simulink model "LunarLandingModel"  (R2023b)
settings: Solver=VariableStepAuto  StartTime=0.0  StopTime=10  RelTol=1e-3
values from neighbouring files (symbols this model uses):
  rf = paramat.rf    [Differential_Eq.m]    (also in control_law.m; extractparameters.m = 1740000; rk4_method.m)
libraries: simulink x1
settings Model: Creator=HUAWEI  LastModifiedBy=HUAWEI

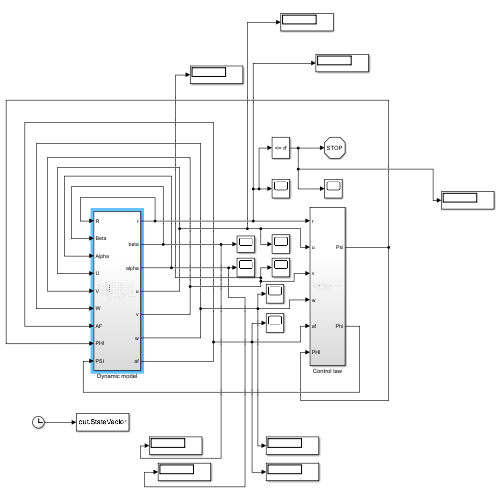
[thumbnail: Simulink's stored preview of the top-level diagram]
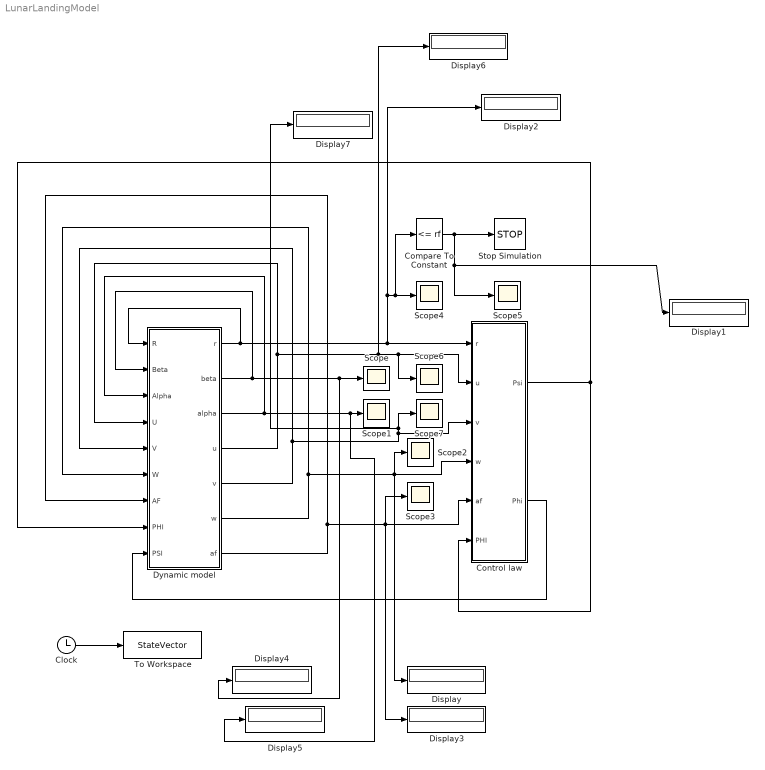
== system LunarLandingModel ==
  Clock : Clock
  Compare To Constant : simulink/Logic and Bit Operations/Compare To Constant  relop=<=  const=rf  OutDataTypeStr=boolean
  Control law : Subsystem
  Display{,1..7} (8 alike) : Display
  Dynamic model : Subsystem
  Scope{,1..7} (8 alike) : Scope
  Stop Simulation : Stop
  To Workspace : ToWorkspace  VariableName=StateVector  SaveFormat=Structure With Time  SampleTime=-1
  wires:
  Dynamic model/1(r) -> Dynamic model/1(R), Display2/1, Compare To Constant/1, Scope4/1, Control law/1(r)
  Dynamic model/2(beta) -> Dynamic model/2(Beta), Scope/1, Display4/1
  Dynamic model/3(alpha) -> Display5/1, Scope1/1, Dynamic model/3(Alpha)
  Compare To Constant/1 -> Scope5/1, Display1/1, Stop Simulation/1
  Clock/1 -> To Workspace/1
  Dynamic model/4(u) -> Control law/2(u), Scope6/1, Display6/1, Dynamic model/4(U)
  Dynamic model/5(v) -> Dynamic model/5(V), Display7/1, Scope7/1, Control law/3(v)
  Dynamic model/6(w) -> Dynamic model/6(W), Display/1, Scope2/1, Control law/4(w)
  Control law/2(Phi) -> Dynamic model/9(PSI)
  Control law/1(Psi) -> Control law/6(PHI), Dynamic model/8(PHI)
  Dynamic model/7(af) -> Dynamic model/7(AF), Display3/1, Scope3/1, Control law/5(af)

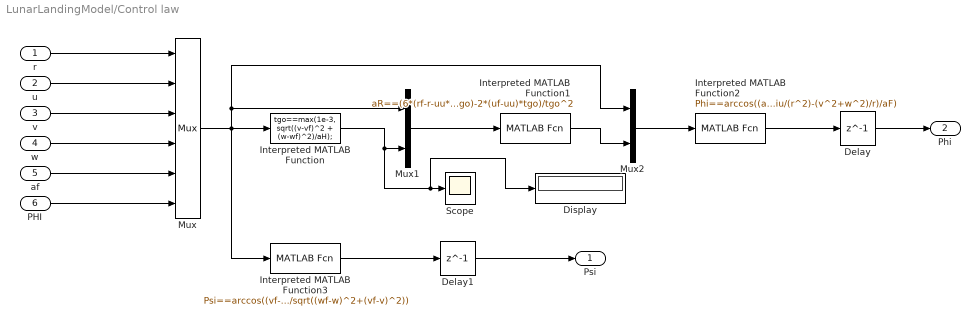
== system LunarLandingModel/Control law ==
  r : Inport
  u : Inport  Port=2
  v : Inport  Port=3
  w : Inport  Port=4
  af : Inport  Port=5
  PHI : Inport  Port=6
  Delay : Delay  DelayLength=1
  Delay1 : Delay  DelayLength=1
  Display : Display
  Interpreted MATLAB Function : MATLABFcn  MATLABFcn=tgo==max(1e-3, sqrt((v-vf)^2 + (w-wf)^2)/aH);
  Interpreted MATLAB Function1 : MATLABFcn  MATLABFcn=aR==(6*(rf-r-uu*tgo)-2*(uf-uu)*tgo)/tgo^2
  Interpreted MATLAB Function2 : MATLABFcn  MATLABFcn=Phi==arccos((aR+miu/(r^2)-(v^2+w^2)/r)/aF)
  Interpreted MATLAB Function3 : MATLABFcn  MATLABFcn=Psi==arccos((vf-v)/sqrt((wf-w)^2+(vf-v)^2))
  Mux : Mux  Inputs=6
  Mux1 : Mux  Inputs=2
  Mux2 : Mux  Inputs=2
  Scope : Scope
  Psi : Outport
  Phi : Outport  Port=2
  wires:
  r/1 -> Mux/1
  u/1 -> Mux/2
  v/1 -> Mux/3
  w/1 -> Mux/4
  af/1 -> Mux/5
  PHI/1 -> Mux/6
  Delay1/1 -> Psi/1
  Interpreted MATLAB Function3/1 -> Delay1/1
  Mux/1 -> Mux2/1, Mux1/1, Interpreted MATLAB Function3/1, Interpreted MATLAB Function/1
  Interpreted MATLAB Function/1 -> Mux1/2, Display/1, Scope/1
  Mux1/1 -> Interpreted MATLAB Function1/1
  Interpreted MATLAB Function1/1 -> Mux2/2
  Mux2/1 -> Interpreted MATLAB Function2/1
  Interpreted MATLAB Function2/1 -> Delay/1
  Delay/1 -> Phi/1

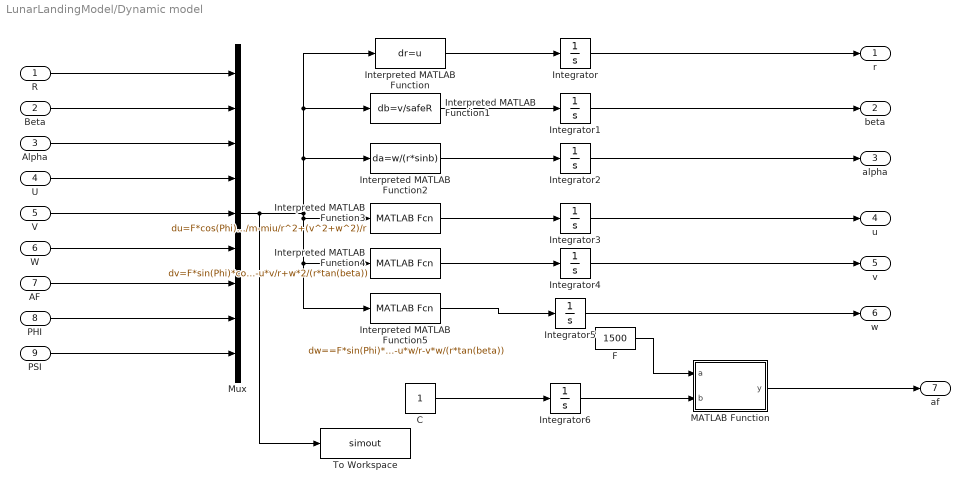
== system LunarLandingModel/Dynamic model ==
  R : Inport
  Beta : Inport  Port=2
  Alpha : Inport  Port=3
  U : Inport  Port=4
  V : Inport  Port=5
  W : Inport  Port=6
  AF : Inport  Port=7
  PHI : Inport  Port=8
  PSI : Inport  Port=9
  C : Constant
  F : Constant  Value=1500
  Integrator : Integrator  InitialCondition=1753e3
  Integrator{1,3,5..6} (4 alike) : Integrator
  Integrator2 : Integrator  InitialCondition=deg2rad(5)
  Integrator4 : Integrator  InitialCondition=1692
  Interpreted MATLAB Function : MATLABFcn  MATLABFcn=dr=u
  Interpreted MATLAB Function1 : MATLABFcn  MATLABFcn=db=v/safeR
  Interpreted MATLAB Function2 : MATLABFcn  MATLABFcn=da=w/(r*sinb)
  Interpreted MATLAB Function3 : MATLABFcn  MATLABFcn=du=F*cos(Phi)/m-miu/r^2+(v^2+w^2)/r
  Interpreted MATLAB Function4 : MATLABFcn  MATLABFcn=dv=F*sin(Phi)*cos(Phi)/m-u*v/r+w*2/(r*tan(beta))
  Interpreted MATLAB Function5 : MATLABFcn  MATLABFcn=dw==F*sin(Phi)*sin(Psi)/m-u*w/r-v*w/(r*tan(beta))
  MATLAB Function : MATLAB Function  TreatAsAtomicUnit=on
  Mux : Mux  Inputs=9
  To Workspace : ToWorkspace  VariableName=simout  SaveFormat=Timeseries  SampleTime=-1
  r : Outport
  beta : Outport  Port=2
  alpha : Outport  Port=3
  u : Outport  Port=4
  v : Outport  Port=5
  w : Outport  Port=6
  af : Outport  Port=7
  wires:
  Integrator/1 -> r/1
  Integrator1/1 -> beta/1
  Integrator2/1 -> alpha/1
  Integrator3/1 -> u/1
  Integrator4/1 -> v/1
  Integrator5/1 -> w/1
  PHI/1 -> Mux/8
  R/1 -> Mux/1
  AF/1 -> Mux/7
  W/1 -> Mux/6
  V/1 -> Mux/5
  Alpha/1 -> Mux/3
  Beta/1 -> Mux/2
  Mux/1 -> To Workspace/1, Interpreted MATLAB Function3/1, Interpreted MATLAB Function4/1, Interpreted MATLAB Function5/1, Interpreted MATLAB Function2/1, Interpreted MATLAB Function1/1, Interpreted MATLAB Function/1
  U/1 -> Mux/4
  PSI/1 -> Mux/9
  Interpreted MATLAB Function/1 -> Integrator/1
  Interpreted MATLAB Function1/1 -> Integrator1/1
  Interpreted MATLAB Function2/1 -> Integrator2/1
  Interpreted MATLAB Function3/1 -> Integrator3/1
  Interpreted MATLAB Function4/1 -> Integrator4/1
  Interpreted MATLAB Function5/1 -> Integrator5/1
  C/1 -> Integrator6/1
  MATLAB Function/1(y) -> af/1
  F/1 -> MATLAB Function/1(a)
  Integrator6/1 -> MATLAB Function/2(b)

== matlab function LunarLandingModel/Dynamic model/MATLAB Function ==
  data: a input; y output; b input
function y = safe_divide(a, b)
    b = max(abs(b), 1e-6) .* sign(b);  % Avoid division by zero
    y = a ./ b;
end
